simulink model "My_gfm_battery_sil_1_PPC2"  (R2018b)
settings: Solver=ode45  StartTime=0.0  StopTime=30  MaxStep=1e-4  RelTol=1e-3
PreLoadFcn:
  | modelDir = fileparts(get_param(bdroot,'FileName'));
  | 
  | load_system(fullfile(modelDir,'controls_element_lib.slx'));
  | load_system(fullfile(modelDir,'test_sequence_lib.slx'));
InitFcn:
  | close all;
  | clear all;
  | clc;
  | 
  | % frequency nominals
  | F_NOM = 60;
  | W_NOM = 2 * pi * F_NOM;
  | 
  | % base values relative to inverter
  | % --------------------------------
  | VLL_INV_NOM = 480;
  | P_INV_NOM = 1e6;
  | Q_INV_NOM = 0.5e6;
  | S_INV_NOM = sqrt(P_INV_NOM^2 + Q_INV_NOM^2);
  | 
  | I_INV_BASE = S_INV_NOM/(sqrt(3)*VLL_INV_NOM);
  | Z_INV_BASE = VLL_INV_NOM^2/S_INV_NOM;
  | L_INV_BASE = Z_INV_BASE / W_NOM;
  | C_INV_BASE = 1 / (Z_INV_BASE * W_NOM);
  | 
  | % nominal ratings for power system model
  | % --------------------------------------
  | INVERTER_COUNT = 100;
  | 
  | VLV_NOM = VLL_INV_NOM;
  | VMV_NOM = 35e3;
  | VHV_NOM = 230e3;
  | S_PLANT = INVERTER_COUNT * S_INV_NOM;
  | 
  | N_GSU = VHV_NOM/VMV_NOM;
  | N_MVT = VMV_NOM/VLV_NOM;
  | 
  | I_LV_BASE = S_PLANT/(sqrt(3)*VLV_NOM);
  | I_MV_BASE = S_PLANT/(sqrt(3)*VMV_NOM);
  | I_HV_BASE = S_PLANT/(sqrt(3)*VHV_NOM);
  | 
  | Z_LV_BASE = VLV_NOM^2/S_PLANT;
  | Z_MV_BASE = VMV_NOM^2/S_PLANT;
  | Z_HV_BASE = VHV_NOM^2/S_PLANT;
  | 
  | L_LV_BASE = Z_LV_BASE / W_NOM;
  | L_MV_BASE = Z_MV_BASE / W_NOM;
  | L_HV_BASE = Z_HV_BASE / W_NOM;
  | C_LV_BASE = 1 / (Z_LV_BASE * W_NOM);
  | C_MV_BASE = 1 / (Z_MV_BASE * W_NOM);
  | C_HV_BASE = 1 / (Z_HV_BASE * W_NOM);
undefined symbols (not defined in the file): dQmax, dQmin, dVmax, dVmin, j, vmax, vmin
libraries: simulink x54, test_sequence_lib x22, controls_element_lib x9
(part 1 of 7)
settings Model: SimulationMode=accelerator  Creator=HussamAlatrash  LastModifiedBy=ahhei
settings SolverCC: ZeroCrossAlgorithm=Adaptive
settings DataIOCC: ReturnWorkspaceOutputs=on
settings OptimizationCC: EfficientMapNaN2IntZero=off
settings DebuggingCC: IgnoredZcDiagnostic=none  UnconnectedInputMsg=none  UnconnectedOutputMsg=none  UnconnectedLineMsg=none
settings HardwareCC: TargetBitPerPointer=64  TargetBitPerSizeT=64  TargetBitPerPtrDiffT=64  TargetLongLongMode=on  TargetIntDivRoundTo=Zero  TargetEndianess=LittleEndian  TargetWordSize=64  TargetHWDeviceType=MATLAB Host  ProdEqTarget=off
settings ModelReferenceCC: EnableRefExpFcnMdlSchedulingChecks=off
settings CodeAppCC: MaxIdLength=128
settings GRTTargetCC: TargetLangStandard=C89/C90 (ANSI)  CombineOutputUpdateFcns=off  GRTInterface=on

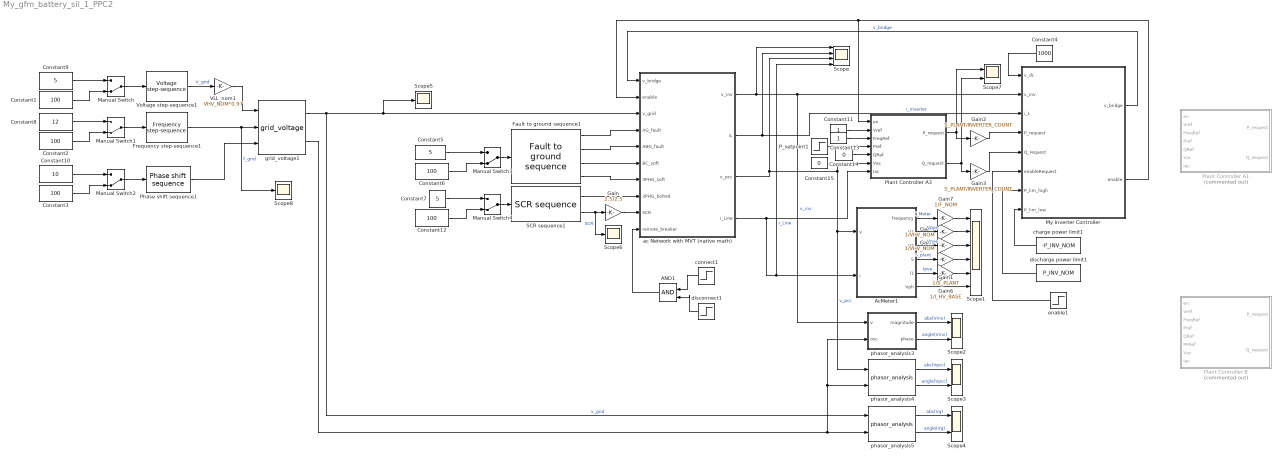
== system My_gfm_battery_sil_1_PPC2 ==
  AND1 : Logic  IconShape=distinctive  AllPortsSameDT=off  OutDataTypeStr=boolean
  AcMeter1 : Subsystem  AncestorBlock=test_sequence_lib/AcMeter  mask{VllRated=VHV_NOM}
      mask prompts: VllRated "Rated line voltage"
  Constant{1..3,6,12} (5 alike) : Constant  Value=100
  Constant10 : Constant  Value=10
  Constant11 : Constant
  Constant13 : Constant
  Constant14 : Constant  Value=0
  Constant15 : Constant  Value=0
  Constant4 : Constant  Value=1000
  Constant5 : Constant  Value=5
  Constant7 : Constant  Value=5
  Constant8 : Constant  Value=12
  Constant9 : Constant  Value=5
  Fault to ground sequence1 : test_sequence_lib/Fault to ground sequence  SystemSampleTime=-1
  Frequency step-sequence1 : test_sequence_lib/Frequency step-sequence  SystemSampleTime=-1
  Gain : Gain  Gain=2.5/2.5
  Gain1 : Gain  Gain=1/S_PLANT
  Gain2 : Gain  Gain=S_PLANT/INVERTER_COUNT
  Gain3 : Gain  Gain=S_PLANT/INVERTER_COUNT
  Gain4 : Gain  Gain=1/VHV_NOM
  Gain5 : Gain  Gain=1/VHV_NOM
  Gain6 : Gain  Gain=1/I_HV_BASE
  Gain7 : Gain  Gain=1/F_NOM
  Manual Switch{,1..4} (5 alike) : ManualSwitch  CurrentSetting=0
  "My Inverter Controller " : Subsystem
  P_setpoint1 : Step  Time=4  After=0.5  SampleTime=0
  Phase shift sequence1 : test_sequence_lib/Phase shift sequence  SystemSampleTime=-1
  Plant Controller A1 : Subsystem  Commented=on  mask(Renewable Energy Plant Controller (REPC_A)){Tfltr=0.02, Xc=0, Rc=0, Kc=0.04, db1=0, emax=0.2, emin=-0.2, Kp=1, Ki=5, Qmax=0.5, Qmin=-0.5, QRefmax=0.5, QRefmin=-0.5, Vfrz=0.8, Tft=0, Tfv=0.1, Vmax=1.05, Vmin=0.95, VcompMode=0, RPCMode=1, fdbd1=0.01*0, fdbd2=-0.01*0, Ddn=20, Dup=20, Tp=0.25, femax=1, femin=-1, Kpg=1, Kig=2, Tlag=0.2, Pmax=1.1, Pmin=-1.1, PRefmax=1, PRefmin=-1, Fmax=1.02, Fmin=-1.02, APCMode=1}
      mask prompts: Tfltr "Voltage/Reactive Power Time Constants [s]"; Xc "Line drop compensation reactance [pu]"; Rc "Line drop compensation resistance [pu]"; Kc "Reactive droop [pu]"; db1 "Reactive power deadline [pu]"; emax "Maximum Volt/VAR error [pu]"; emin "Minimum Volt/VAR error [pu]"; Kp "Volt/VAR Propotional Gain [pu/pu]"; Ki "Volt/VAR Integral Gain [pu/pu-s]"; Qmax "Max Cmd Reactive Power [pu]"; Qmin "Min Cmd Reactive Power [pu]"; QRefmax "Max Ref Reactive Power [pu]"; QRefmin "Min Ref Reactive Power [pu]"; Vfrz "Voltage for Freezing Volt/VAR Integrator [pu]"; Tft "Q Lead Time Constant [s]"; Tfv "Q Lag Time Constant [s]"; Vmax "Maximun Voltage Reference [pu]"; Vmin "Minimum Voltage Reference [pu]"; VcompMode "Voltage Compensation Mode"; RPCMode "Reactive Power Control Mode"; fdbd1 "Overfrequency deadband for govenor [pu]"; fdbd2 "Underfrequency deadband for govenor [pu]"; Ddn "Down regulation droop [pu]"; Dup "Up regulation droop [pu]"; Tp "Active Power Filter Time Constant [s]"; femax "Maximum Power Error [pu]"; femin "Minimum Power Error [pu]"; Kpg "Active Power regulator gain [pu]"; Kig "Active Power integral gain [pu]"; Tlag "Plant Controller P output Lag [s]"; Pmax "Maximum Cmd Active Power [pu]"; Pmin "Minimum Cmd Active Power [pu]"; PRefmax "Maximum Ref Active Power [pu]"; PRefmin "Minimum Ref Active Power [pu]"; Fmax "Maximum Frequency Reference [pu]"; Fmin "Minimum Frequency Reference [pu]"; APCMode "Active Power Control Mode"
      mask DialogControl Container3 Prompt: Reactive Power Control
      mask DialogControl Container4 Prompt: Active Power Control
  Plant Controller A3 : Subsystem  mask(Renewable Energy Plant Controller (REPC_A)){Tfltr=0.02, Xc=0, Rc=0, Kc=0.04, db1=0, emax=0.2, emin=-0.2, Kp=1, Ki=5, Qmax=0.5, Qmin=-0.5, QRefmax=0.5, QRefmin=-0.5, Vfrz=0.8, Tft=0, Tfv=0.1, Vmax=1.05, Vmin=0.95, VcompMode=0, RPCMode=1, fdbd1=0.01*0, fdbd2=-0.01*0, Ddn=20, Dup=20, Tp=0.25, femax=1, femin=-1, Kpg=1, Kig=2, Tlag=0.2, Pmax=1.1, Pmin=-1.1, PRefmax=1, PRefmin=-1, Fmax=1.02, Fmin=-1.02, APCMode=1}
      mask prompts: Tfltr "Voltage/Reactive Power Time Constants [s]"; Xc "Line drop compensation reactance [pu]"; Rc "Line drop compensation resistance [pu]"; Kc "Reactive droop [pu]"; db1 "Reactive power deadline [pu]"; emax "Maximum Volt/VAR error [pu]"; emin "Minimum Volt/VAR error [pu]"; Kp "Volt/VAR Propotional Gain [pu/pu]"; Ki "Volt/VAR Integral Gain [pu/pu-s]"; Qmax "Max Cmd Reactive Power [pu]"; Qmin "Min Cmd Reactive Power [pu]"; QRefmax "Max Ref Reactive Power [pu]"; QRefmin "Min Ref Reactive Power [pu]"; Vfrz "Voltage for Freezing Volt/VAR Integrator [pu]"; Tft "Q Lead Time Constant [s]"; Tfv "Q Lag Time Constant [s]"; Vmax "Maximun Voltage Reference [pu]"; Vmin "Minimum Voltage Reference [pu]"; VcompMode "Voltage Compensation Mode"; RPCMode "Reactive Power Control Mode"; fdbd1 "Overfrequency deadband for govenor [pu]"; fdbd2 "Underfrequency deadband for govenor [pu]"; Ddn "Down regulation droop [pu]"; Dup "Up regulation droop [pu]"; Tp "Active Power Filter Time Constant [s]"; femax "Maximum Power Error [pu]"; femin "Minimum Power Error [pu]"; Kpg "Active Power regulator gain [pu]"; Kig "Active Power integral gain [pu]"; Tlag "Plant Controller P output Lag [s]"; Pmax "Maximum Cmd Active Power [pu]"; Pmin "Minimum Cmd Active Power [pu]"; PRefmax "Maximum Ref Active Power [pu]"; PRefmin "Minimum Ref Active Power [pu]"; Fmax "Maximum Frequency Reference [pu]"; Fmin "Minimum Frequency Reference [pu]"; APCMode "Active Power Control Mode"
      mask DialogControl Container3 Prompt: Reactive Power Control
      mask DialogControl Container4 Prompt: Active Power Control
  Plant Controller B : Subsystem  Commented=on  mask(Renewable Energy Plant Controller (REPC_A)){Tfltr=0.02, Ts=1e-3, Vfrz=0.8, VcompMode=0, Kc=0.04, Vmax=1.05, Vmin=0.95, Verrmax=0.2, Verrmin=-0.2, vdbd1=0, vdbd2=0, Kpvdn=1, Kpvup=1, Tpv=0.1, Kiv=0, Vleak=10e-3, Vintmax=0.3, Vintmin=-0.3, RPCMode=1, Tpf=0, QRiseRate=1, QFallRate=-1, QRefmax=0.5, QRefmin=-0.5, Kpq=1, Kiq=2, Qleak=10e-3, Qerrmax=0.2, Qerrmin=-0.2, Qintmax=0.3, Qintmin=-0.3, Xc=0, Qmax=0.5, Qmin=-0.5, Tleadq=0, Tlagq=0.1, PRiseRate=1, PFallRate=-1, Fmax=1.05, Fmin=0.95, fdbd1=0.01*0, fdbd2=-0.01*0, Kpfdn=20, Kpfup=20, Pfreqmax=0.5, Pfreqmin=-0.5, Tfp=0.1, FFRLo_en=0, FFRThresLo=58.5/60, FFRTrigLoTime=0.2, FFRRestLo_en=0, FFRRestThresLo=59.5/60, FFRRestLoTime=0.2, FFRHoldLoTime=5, FFRPowerLo=0.5, FFRLoRiseRate=1, FFRLoFallRate=-1, Time1=0, FFRHi_en=0, FFRThresHi=61.5/60, FFRTrigHiTime=0.2, FFRRestHi_en=0, FFRRestThresHi=60.5/60, FFRRestHiTime=0.2, FFRHoldHiTime=5, FFRPowerHi=-0.5, FFRHiRiseRate=1, FFRHiFallRate=-1, Time2=0, PRefmax=1, PRefmin=-1, Tp=0.02, Kpp=1, Kip=2, Pleak=10e-3, Perrmax=0.2, Perrmin=-0.2, Pintmax=0.3, Pintmin=-0.3, APCMode=1, Rc=0, Pmax=1.1, Pmin=-1.1, Tlagp=0.2}
      mask prompts: Tfltr "Voltage/Reactive Power Time Constants [s]"; Ts "Time Step"; Vfrz "LVRT Threshold Voltage [pu]"; VcompMode "Voltage Compensation Mode"; Kc "Reactive droop [pu]"; Vmax "Maximum Voltage Reference [pu]"; Vmin "Minimum Voltage Reference [pu]"; Verrmax "Maximum Voltage Error  [pu]"; Verrmin "Minimum Voltage Error  [pu]"; vdbd1 "Voltage HiDeadband [pu]"; vdbd2 "Voltage LoDeadband [pu]"; Kpvdn "Voltage Down Proportional Gain [pu]"; Kpvup "Voltage Up Proportional Gain [pu]"; Tpv "Voltage Proportinal LPF Time Constants [s]"; Kiv "Voltage Integral Gain [pu]"; Vleak "Voltage Integral Leak Gain [pu]"; Vintmax "Maximum Voltage Integrator error [pu]"; Vintmin "Minimum Voltage Integrator error [pu]"; RPCMode "Reactive Power Control Mode"; Tpf "Power Factor LPF Time Constants [s]"; QRiseRate "Reactive Power Reference Rise Ramp Rate [pu/s]"; QFallRate "Reactive Power Reference Fall Ramp Rate [pu/s]"; QRefmax "Max Ref Reactive Power [pu]"; QRefmin "Min Ref Reactive Power [pu]"; Kpq "Reactive Power Propotional Gain [pu]"; Kiq "Reactive Power Integral Gain [pu]"; Qleak "Reactive Power Integral Leak Gain [pu]"; Qerrmax "Maximum Reactive Power error [pu]"; Qerrmin "Minimum Reactive Power error [pu]"; Qintmax "Maximum Reactive Power Integrator error [pu]"; Qintmin "Minimum Reactive Power Integrator error [pu]"; Xc "Loss compensation reactance [pu]"; Qmax "Max Cmd Reactive Power [pu]"; Qmin "Min Cmd Reactive Power [pu]"; Tleadq "Reactive Power Output Lead Time Constant [s]"; Tlagq "Reactive Power Output Lag Time Constant [s]"; PRiseRate "Active Power Reference Rise Ramp Rate [pu/s]"; PFallRate "Active Power Reference Fall Ramp Rate [pu/s]"; Fmax "Maximum Frequency Reference [pu]"; Fmin "Minimum Frequency Reference [pu]"; fdbd1 "Frequency HiDeadband [pu]"; fdbd2 "Frequency Lodeadband [pu]"; Kpfdn "Frequency Down Proportional Gain [pu]"; Kpfup "Frequency Up Proportional Gain [pu]"; Pfreqmax "Maximum Frequency Power [pu]"; Pfreqmin "Minimum Frequency Power [pu]"; Tfp "Frequency Power Proportinal LPF Time Constants [s]"; FFRLo_en "Enable Under Frequency FFR"; FFRThresLo "Trigger Threshold [pu]"; FFRTrigLoTime "Trigger Qualification Time [sec]"; FFRRestLo_en "Enable Restore Threshold"; FFRRestThresLo "Restore Threshold [pu]"; FFRRestLoTime "Restore Qualification Time [sec]"; FFRHoldLoTime "Hold Time [sec]"; FFRPowerLo "Power Response [pu]"; FFRLoRiseRate "Power Response Rise Rate [pu/s]"; FFRLoFallRate "Power Response Fall Rate [pu/s]"; Time1 "Condition Clear Time [sec]"; FFRHi_en "Enable Under Frequency FFR"; FFRThresHi "Trigger Threshold [pu]"; FFRTrigHiTime "Trigger Qualification Time [sec]"; FFRRestHi_en "Enable RestoreThreshold"; FFRRestThresHi "Restore Threshold [pu]"; FFRRestHiTime "Restore Qualification Time [sec]"; FFRHoldHiTime "Hold Time [sec]"; FFRPowerHi "Power Response [pu]"; FFRHiRiseRate "Power Response Rise Rate [pu/s]"; FFRHiFallRate "Power Response Fall Rate [pu/s]"; Time2 "Condition Clear Time [sec]"; PRefmax "Maximum Ref Active Power [pu]"; PRefmin "Minimum Ref Active Power [pu]"; Tp "Active Power Filter Time Constant [s]"; Kpp "Active Power Propotional Gain [pu]"; Kip "Active Power Integral Gain [pu]"; Pleak "Active Power Integral Leak Gain [pu]"; Perrmax "Maximum Active Power error [pu]"; Perrmin "Minimum Active Power error [pu]"; Pintmax "Maximum Active Power Integrator error [pu]"; Pintmin "Minimum Active Power Integrator error [pu]"; APCMode "Active Power Control Mode"; Rc "Loss compensation resistance [pu]"; Pmax "Maximum Cmd Active Power [pu]"; Pmin "Minimum Cmd Active Power [pu]"; Tlagp "Active Power Output Lag Time Constant [s]"
      mask DialogControl Container15 Prompt: Reactive Power Path
      mask DialogControl Container3 Prompt: Voltage/Reactive Power Control
      mask DialogControl Container5 Prompt: Voltage Control
      mask DialogControl Container6 Prompt: Reactive Power Control
      mask DialogControl Container20 Prompt: Active Power Path
      mask DialogControl Container4 Prompt: Reference and Control
      mask DialogControl Container9 Prompt: Active Power Reference
      mask DialogControl Container10 Prompt: Frequency Control
      mask DialogControl Container11 Prompt: Primary Frequency Response
      mask DialogControl Container13 Prompt: Fast Frequency Response
      mask DialogControl Container16 Prompt: Under Frequency FFR
      mask DialogControl Container16_copy Prompt: Over Frequency FFR
      mask DialogControl Container8 Prompt: Active Power Control
  SCR sequence1 : test_sequence_lib/SCR sequence  SystemSampleTime=-1
  Scope : Scope  NumInputPorts=4
  Scope1 : Scope  NumInputPorts=6
  Scope{2..4,7} (4 alike) : Scope  NumInputPorts=2
  Scope5 : Scope
  Scope6 : Scope
  Scope8 : Scope
  VLL_nom1 : Gain  Gain=VHV_NOM*0.97
  Voltage step-sequence1 : test_sequence_lib/Voltage step-sequence  SystemSampleTime=-1
  ac Network with MVT (native math) : Subsystem  AncestorBlock=test_sequence_lib/ac Network with MVT (native math)
  charge power limit1 : Constant  Value=-P_INV_NOM
  connect1 : Step  Time=0  SampleTime=0
  discharge power limit1 : Constant  Value=P_INV_NOM
  disconnect1 : Step  Time=100  Before=1  After=0  SampleTime=0
  enable1 : Step  Time=0.5  SampleTime=0
  grid_voltage1 : test_sequence_lib/grid_voltage  SystemSampleTime=-1
  phasor_analysis3 : Subsystem  AncestorBlock=test_sequence_lib/phasor_analysis
  phasor_analysis4 : test_sequence_lib/phasor_analysis  SystemSampleTime=-1
  phasor_analysis5 : test_sequence_lib/phasor_analysis  SystemSampleTime=-1
  wires:
  Voltage step-sequence1/1 -> VLL_nom1/1  "V_grid"
  Manual Switch/1 -> Voltage step-sequence1/1
  Fault to ground sequence1/2 -> ac Network with MVT (native math)/5(ABG_fault)
  AND1/1 -> ac Network with MVT (native math)/10(remote_breaker)
  Constant4/1 -> "My Inverter Controller "/1(v_dc)
  AcMeter1/3(V2) -> Gain5/1  "Vnve"
  discharge power limit1/1 -> "My Inverter Controller "/7(P_lim_high)
  Fault to ground sequence1/3 -> ac Network with MVT (native math)/6(BC_soft)
  AcMeter1/6(Vph) -> Scope1/6
  "My Inverter Controller "/1(v_bridge) -> ac Network with MVT (native math)/1(v_bridge)  "v_bridge"
  AcMeter1/2(V1) -> Gain4/1  "Vpve"
  Plant Controller A3/1(P_request) -> Gain2/1, Scope7/1
  ac Network with MVT (native math)/1(v_inv) -> phasor_analysis3/1(v), "My Inverter Controller "/2(v_inv), Scope/1  "v_inv"
  phasor_analysis5/1 -> Scope4/1  "abs(Vg)"
  AcMeter1/5(I1) -> Gain6/1  "Ipve"
  Plant Controller A3/2(Q_request) -> Gain3/1, Scope7/2
  grid_voltage1/1 -> phasor_analysis5/1, Scope5/1, ac Network with MVT (native math)/3(v_grid)  "v_grid"
  SCR sequence1/1 -> ac Network with MVT (native math)/8(3PHG_bolted)
  phasor_analysis3/1(magnitude) -> Scope2/1  "abs(Vinv)"
  AcMeter1/4(S) -> Gain1/1  "S_plant"
  ac Network with MVT (native math)/4(i_Line) -> Plant Controller A3/7(Iac), Scope/4, AcMeter1/2(i)  "i_Line"
  AcMeter1/1(frequency) -> Gain7/1  "f_Meter"
  VLL_nom1/1 -> grid_voltage1/1
  phasor_analysis3/2(phase) -> Scope2/2  "angle(Vinv)"
  SCR sequence1/2 -> Scope6/1, Gain/1  "SCR"
  ac Network with MVT (native math)/2(iL) -> "My Inverter Controller "/3(i_L), Scope/2  "i_inverter"
  disconnect1/1 -> AND1/2
  Fault to ground sequence1/4 -> ac Network with MVT (native math)/7(3PHG_soft)
  ac Network with MVT (native math)/3(v_pcc) -> Plant Controller A3/6(Vac), phasor_analysis4/1, AcMeter1/1(v), Scope/3  "v_pcc"
  charge power limit1/1 -> "My Inverter Controller "/8(P_lim_low)
  "My Inverter Controller "/2(enable) -> Plant Controller A3/1(en), ac Network with MVT (native math)/2(enable)
  Frequency step-sequence1/1 -> Scope8/1, grid_voltage1/2  "f_grid"
  Fault to ground sequence1/1 -> ac Network with MVT (native math)/4(AG_fault)
  grid_voltage1/2 -> phasor_analysis4/2, phasor_analysis3/2(osc), phasor_analysis5/2
  phasor_analysis5/2 -> Scope4/2  "angle(Vg)"
  enable1/1 -> "My Inverter Controller "/6(enableRequest)
  connect1/1 -> AND1/1
  Constant9/1 -> Manual Switch/1
  Constant1/1 -> Manual Switch/2
  Constant2/1 -> Manual Switch1/2
  Manual Switch1/1 -> Frequency step-sequence1/1
  Constant8/1 -> Manual Switch1/1
  Manual Switch2/1 -> Phase shift sequence1/1
  Constant3/1 -> Manual Switch2/2
  Constant10/1 -> Manual Switch2/1
  Constant6/1 -> Manual Switch3/2
  Constant5/1 -> Manual Switch3/1
  Manual Switch3/1 -> Fault to ground sequence1/1
  Constant7/1 -> Manual Switch4/1
  Constant12/1 -> Manual Switch4/2
  Manual Switch4/1 -> SCR sequence1/1
  phasor_analysis4/1 -> Scope3/1  "abs(Vpcc)"
  phasor_analysis4/2 -> Scope3/2  "angle(Vpcc)"
  Phase shift sequence1/1 -> grid_voltage1/3
  Gain2/1 -> "My Inverter Controller "/4(P_request)
  Gain3/1 -> "My Inverter Controller "/5(Q_request)
  Gain/1 -> ac Network with MVT (native math)/9(SCR)
  Gain1/1 -> Scope1/4
  Gain4/1 -> Scope1/2
  Gain5/1 -> Scope1/3
  Gain6/1 -> Scope1/5
  Gain7/1 -> Scope1/1
  Constant11/1 -> Plant Controller A3/2(Vref)
  Constant13/1 -> Plant Controller A3/3(FreqRef)
  P_setpoint1/1 -> Plant Controller A3/4(Pref)
  Constant14/1 -> Plant Controller A3/5(QRef)

== system My_gfm_battery_sil_1_PPC2/AcMeter1 ==
  note: in pu:
      | S = sqrt(3) * VLL * conj(I)
  v : Inport
  i : Inport  Port=2
  Complex to Magnitude : ComplexToMagnitudeAngle  Output=Magnitude
  Complex to Magnitude1 : ComplexToMagnitudeAngle  Output=Magnitude
  Complex to Magnitude2 : ComplexToMagnitudeAngle  Output=Magnitude
  Conj : Math  Operator=conj  SaturateOnIntegerOverflow=on
  PLL_3ph : Subsystem
  Product : Product
  RMS calculator : Subsystem
  Sum of Elements : Sum  Inputs=+
  Terminator : Terminator
  Terminator1 : Terminator
  Terminator2 : Terminator
  overVnom : Gain  Gain=1/VllRated
  phasor_analysis : Subsystem
  phasor_analysis1 : Subsystem  AncestorBlock=test_sequence_lib/AcMeter/phasor_analysis
  sqrt(3) : Gain  Gain=sqrt(3)
  sqrt(3)1 : Gain  Gain=sqrt(3)
  sqrt(3)2 : Gain  Gain=sqrt(3)
  frequency : Outport  VectorParamsAs1DForOutWhenUnconnected=on
  V1 : Outport  Port=2  VectorParamsAs1DForOutWhenUnconnected=on
  V2 : Outport  Port=3  VectorParamsAs1DForOutWhenUnconnected=on
  S : Outport  Port=4  VectorParamsAs1DForOutWhenUnconnected=on
  I1 : Outport  Port=5  VectorParamsAs1DForOutWhenUnconnected=on
  Vph : Outport  Port=6  VectorParamsAs1DForOutWhenUnconnected=on
  wires:
  RMS calculator/1(out[3]) -> Vph/1
  PLL_3ph/2(osc[3]) -> phasor_analysis/2(osc), phasor_analysis1/2(osc)
  Sum of Elements/1 -> S/1  "S"
  v/1 -> RMS calculator/1(in[3]), phasor_analysis/1(in), overVnom/1
  PLL_3ph/1(freq) -> frequency/1
  overVnom/1 -> PLL_3ph/1(ref)
  Conj/1 -> Product/2
  Product/1 -> Sum of Elements/1
  phasor_analysis/2(pve) -> sqrt(3)/1  "Vpve_LN"
  phasor_analysis/3(nve) -> sqrt(3)1/1
  phasor_analysis1/2(pve) -> Complex to Magnitude2/1, Conj/1  "Ipve"
  sqrt(3)1/1 -> Complex to Magnitude1/1  "Vnve_LL"
  i/1 -> phasor_analysis1/1(in)
  sqrt(3)/1 -> Complex to Magnitude/1, sqrt(3)2/1  "Vpve_LL"
  sqrt(3)2/1 -> Product/1
  phasor_analysis/1(perPh) -> Terminator/1
  phasor_analysis1/1(perPh) -> Terminator1/1
  phasor_analysis1/3(nve) -> Terminator2/1
  Complex to Magnitude/1 -> V1/1  "Ve"
  Complex to Magnitude1/1 -> V2/1  "Ve"
  Complex to Magnitude2/1 -> I1/1  "Ve"

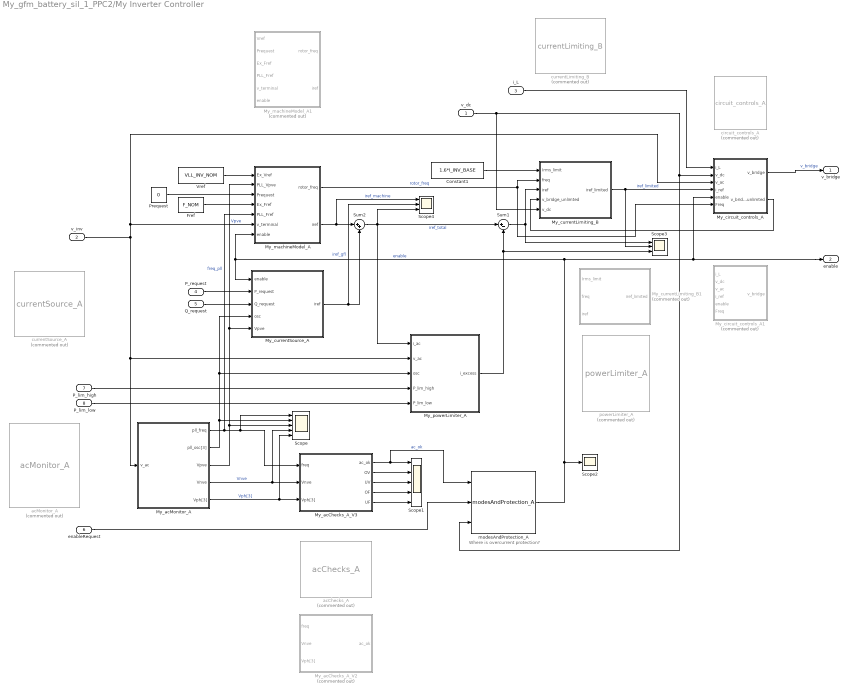
== system My_gfm_battery_sil_1_PPC2/My Inverter Controller  ==
  note: Where is overcurrent protection?
  v_dc : Inport
  v_inv : Inport  Port=2
  i_L : Inport  Port=3
  P_request : Inport  Port=4
  Q_request : Inport  Port=5
  enableRequest : Inport  Port=6
  P_lim_high : Inport  Port=7
  P_lim_low : Inport  Port=8
  Constant1 : Constant  Value=1.6*I_INV_BASE
  Fref : Constant  Value=F_NOM
  My_acChecks_A_V2 : Subsystem  Commented=on  AncestorBlock=controls_element_lib/acChecks_A  mask{VllRated=VLL_INV_NOM, NominalFrequency=F_NOM, Ts=1e-3, Time1=2, Time2=0, VHi=1.15, VLo=0.85, FHi=62, FLo=58, VNeg=0.2, Time3=0, OV3=1.3, OV3_Time=0.02, OV3_en=1, OV2=1.25, OV2_Time=2, OV2_en=1, OV1=1.2, OV1_Time=20, OV1_en=1, UV1=0.81, UV1_Time=15, UV1_en=1, UV2=0.5, UV2_Time=5, UV2_en=1, UV3=0.2, UV3_Time=1, UV3_en=1, OF3=70, OF3_Time=0.2, OF3_en=1, OF2=65, OF2_Time=10, OF2_en=1, OF1=63, OF1_Time=30, OF1_en=1, UF1=56, UF1_Time=30, UF1_en=1, UF2=55, UF2_Time=10, UF2_en=1, UF3=50, UF3_Time=0.2, UF3_en=1}
      mask prompts: VllRated "Rated Line-to-Line Voltage (V)"; NominalFrequency "Nominal Line Frequency (Hz)"; Ts "Operating Sample Time (sec)"; Time1 "Connection Time (sec)"; Time2 "Connection Out-of-Condition Delay (sec)"; VHi "High Voltage Threshold (pu)"; VLo "Low Voltage Threshold (pu)"; FHi "High Frequency Threshold (Hz)"; FLo "Low Frequency Threshold (Hz)"; VNeg "Negative Sequence Voltage Threshold (pu)"; Time3 "Trip Out-of-Condition Delay (sec)"; OV3 "OV PickUp 3 (pu)"; OV3_Time "OV Time 3 (sec)"; OV3_en "OV Enable 3"; OV2 "OV PickUp 2 (pu)"; OV2_Time "OV Time 2 (sec)"; OV2_en "OV Enable 2"; OV1 "OV PickUp 1 (pu)"; OV1_Time "OV Time 1 (sec)"; OV1_en "OV Enable 1"; UV1 "UV PickUp 1 (pu)"; UV1_Time "UV Time 1 (sec)"; UV1_en "UV Enable 1"; UV2 "UV PickUp 2 (pu)"; UV2_Time "UV Time 2 (sec)"; UV2_en "UV Enable 2"; UV3 "UV PickUp 3 (pu)"; UV3_Time "UV Time 3 (sec)"; UV3_en "UV Enable 3"; OF3 "OF PickUp 3 (Hz)"; OF3_Time "OF Time 3 (pu)"; OF3_en "OF Enable 3"; OF2 "OF PickUp 2 (Hz)"; OF2_Time "OF Time 2 (pu)"; OF2_en "OF Enable 2"; OF1 "OF PickUp 1 (Hz)"; OF1_Time "OF Time 1 (pu)"; OF1_en "OF Enable 1"; UF1 "UF PickUp 1 (Hz)"; UF1_Time "UF Time 1 (sec)"; UF1_en "UF Enable 1"; UF2 "UF PickUp 2 (Hz)"; UF2_Time "UF Time 2 (sec)"; UF2_en "UF Enable 2"; UF3 "UF PickUp 3 (Hz)"; UF3_Time "UF Time 3 (sec)"; UF3_en "UF Enable 3"
      mask DialogControl DescGroupVar Prompt: ACChecks
      mask DialogControl DecsTextVar Prompt: Grid Checks for Connection and Tripping
      mask DialogControl ParameterGroupVar Prompt: General Parameters
      mask DialogControl Container11 Prompt: Connection Settings
      mask DialogControl Container20 Prompt: Thresholds
      mask DialogControl Container3 Prompt: Trip Settings
      mask DialogControl Container12 Prompt: General Parameters
      mask DialogControl Container15 Prompt: Over Voltage Settings
      mask DialogControl Container4 Prompt: Over Voltage
      mask DialogControl Container19 Prompt: Under Voltage Settings
      mask DialogControl Container7 Prompt: Under Voltage
      mask DialogControl Container17 Prompt: Over Frequency Settings
      mask DialogControl Container9 Prompt: Over Frequency
      mask DialogControl Container16 Prompt: Under Frequency Settings
      mask DialogControl Container10 Prompt: Under Frequency
  My_acChecks_A_V3 : Subsystem  AncestorBlock=controls_element_lib/acChecks_A  mask{VllRated=VLL_INV_NOM, NominalFrequency=F_NOM, Ts=1e-3, Time1=2, Time2=0, VHi=1.15, VLo=0.85, FHi=62, FLo=58, VNeg=0.2, Time3=0, OV3=1.3, OV3_Time=0.02, OV3_en=1, OV2=1.25, OV2_Time=2, OV2_en=1, OV1=1.2, OV1_Time=20, OV1_en=1, UV1=0.81, UV1_Time=15, UV1_en=1, UV2=0.5, UV2_Time=5, UV2_en=1, UV3=0.2, UV3_Time=1, UV3_en=1, OF3=70, OF3_Time=0.2, OF3_en=1, OF2=65, OF2_Time=10, OF2_en=1, OF1=63, OF1_Time=30, OF1_en=1, UF1=56, UF1_Time=30, UF1_en=1, UF2=55, UF2_Time=10, UF2_en=1, UF3=50, UF3_Time=0.2, UF3_en=1}
      mask prompts: VllRated "Rated Line-to-Line Voltage (V)"; NominalFrequency "Nominal Line Frequency (Hz)"; Ts "Operating Sample Time (sec)"; Time1 "Connection Time (sec)"; Time2 "Connection Out-of-Condition Delay (sec)"; VHi "High Voltage Threshold (pu)"; VLo "Low Voltage Threshold (pu)"; FHi "High Frequency Threshold (Hz)"; FLo "Low Frequency Threshold (Hz)"; VNeg "Negative Sequence Voltage Threshold (pu)"; Time3 "Trip Out-of-Condition Delay (sec)"; OV3 "OV PickUp 3 (pu)"; OV3_Time "OV Time 3 (sec)"; OV3_en "OV Enable 3"; OV2 "OV PickUp 2 (pu)"; OV2_Time "OV Time 2 (sec)"; OV2_en "OV Enable 2"; OV1 "OV PickUp 1 (pu)"; OV1_Time "OV Time 1 (sec)"; OV1_en "OV Enable 1"; UV1 "UV PickUp 1 (pu)"; UV1_Time "UV Time 1 (sec)"; UV1_en "UV Enable 1"; UV2 "UV PickUp 2 (pu)"; UV2_Time "UV Time 2 (sec)"; UV2_en "UV Enable 2"; UV3 "UV PickUp 3 (pu)"; UV3_Time "UV Time 3 (sec)"; UV3_en "UV Enable 3"; OF3 "OF PickUp 3 (Hz)"; OF3_Time "OF Time 3 (pu)"; OF3_en "OF Enable 3"; OF2 "OF PickUp 2 (Hz)"; OF2_Time "OF Time 2 (pu)"; OF2_en "OF Enable 2"; OF1 "OF PickUp 1 (Hz)"; OF1_Time "OF Time 1 (pu)"; OF1_en "OF Enable 1"; UF1 "UF PickUp 1 (Hz)"; UF1_Time "UF Time 1 (sec)"; UF1_en "UF Enable 1"; UF2 "UF PickUp 2 (Hz)"; UF2_Time "UF Time 2 (sec)"; UF2_en "UF Enable 2"; UF3 "UF PickUp 3 (Hz)"; UF3_Time "UF Time 3 (sec)"; UF3_en "UF Enable 3"
      mask DialogControl DescGroupVar Prompt: ACChecks
      mask DialogControl DecsTextVar Prompt: Grid Checks for Connection and Tripping
      mask DialogControl ParameterGroupVar Prompt: General Parameters
      mask DialogControl Container11 Prompt: Connection Settings
      mask DialogControl Container20 Prompt: Thresholds
      mask DialogControl Container3 Prompt: Trip Settings
      mask DialogControl Container12 Prompt: General Parameters
      mask DialogControl Container15 Prompt: Over Voltage Settings
      mask DialogControl Container4 Prompt: Over Voltage
      mask DialogControl Container19 Prompt: Under Voltage Settings
      mask DialogControl Container7 Prompt: Under Voltage
      mask DialogControl Container17 Prompt: Over Frequency Settings
      mask DialogControl Container9 Prompt: Over Frequency
      mask DialogControl Container16 Prompt: Under Frequency Settings
      mask DialogControl Container10 Prompt: Under Frequency
  My_acMonitor_A : Subsystem  AncestorBlock=controls_element_lib/acMonitor_A  mask{VllRated=VLL_INV_NOM, nominalFrequency=F_NOM}
      mask prompts: VllRated "Rated line-to-line voltage (V)"; nominalFrequency "Nominal line frequency (Hz)"
  My_circuit_controls_A : Subsystem  AncestorBlock=controls_element_lib/circuit_controls_A
  My_circuit_controls_A1 : Subsystem  Commented=on  AncestorBlock=controls_element_lib/circuit_controls_A
  My_currentLimiting_B : Subsystem  AncestorBlock=controls_element_lib/currentLimiting_B  mask{IRated=I_INV_BASE, peakSoftLimit=2.6, peakHardLimit=3.6}
      mask prompts: IRated "Rated current (A)"; peakSoftLimit "Soft peak limit (pu)"; peakHardLimit "Hard peak limit (pu)"
  My_currentLimiting_B1 : Subsystem  Commented=on  AncestorBlock=controls_element_lib/currentLimiting_B  mask{IRated=I_INV_BASE, peakSoftLimit=2.6, peakHardLimit=3.6}
      mask prompts: IRated "Rated current (A)"; peakSoftLimit "Soft peak limit (pu)"; peakHardLimit "Hard peak limit (pu)"
  My_currentSource_A : Subsystem  AncestorBlock=controls_element_lib/currentSource_A  mask{VllRated=VLL_INV_NOM, SRated=S_INV_NOM, nominalFrequency=F_NOM, Plimit=P_INV_NOM/S_INV_NOM, Qlimit=Q_INV_NOM/S_INV_NOM, CSOnline=1}
      mask prompts: VllRated "Rated line-to-line voltage (V)"; SRated "Rated power (VA)"; nominalFrequency "Nominal line frequency (Hz)"; Plimit "Real power request limit (pu)"; Qlimit "Reactive power request limit (pu)"; CSOnline "Current Source Online"
  My_machineModel_A : Subsystem  AncestorBlock=controls_element_lib/machineModel_A  mask{SRated=S_INV_NOM, VllRated=VLL_INV_NOM, nominalFrequency=F_NOM, MachOnline=0, inertialConstant=2.5, kDamper=2, tau_damp=0.3, Xs=0.3, rs=0.08, rn=0, wExciter=10, VoltRefSel=0, AVROnline=0, kqDroop=0, Xcomp=0, kp=5, ki=1, leak=10e-3, FreqRefSel=0, kDroop=1, wGoverner=1/0.3, kpSync=20, kpFastSync=1, wSync=2*pi*50, kpSyncFade=4, SyncFadeThres=0.2, tauMeas=0.02, tauBkSt=0.5}
      mask prompts: SRated "Rated power (VA)"; VllRated "Rated Voltage (Volts, line-to-line)"; nominalFrequency "Nominal frequency (Hz)"; MachOnline "Machine Online"; inertialConstant "Inertial constant (seconds)"; kDamper "Damper gain (pu/Hz)"; tau_damp "Damper time constant (sec)"; Xs "Stator reactance (pu)"; rs "Stator resistance (pu)"; rn "Neutral resistance (pu)"; wExciter "Exciter Bandwidth (rad)"; VoltRefSel "Voltage Reference Selector"; AVROnline "AVR Online"; kqDroop "QV Droop (pu v/ pu Q)"; Xcomp "Line drop compensation (pu)"; kp "Proportional gain"; ki "Integral gain"; leak "Leakage"; FreqRefSel "Frequency Reference Selector"; kDroop "Droop gain (pu/Hz)"; wGoverner "Governer Bandwidth (rad/s)"; kpSync "Synchronizer proportional gain (pu P / pu V)"; kpFastSync "Fast synchronizer gain (pu P / pu V)"; wSync "Synchronizer HPF Bandwidth(rad/s)"; kpSyncFade "Synchronizer fade gain (pu P/ puV)"; SyncFadeThres "Synchronizer fade threshold (pu)"; tauMeas "Measurements filters time constant (sec)"; tauBkSt "Black Start filter time constant (sec)"
      mask DialogControl DescGroupVar Prompt: Machine Model and Controls
      mask DialogControl ParameterGroupVar Prompt: Ratings
      mask DialogControl Container3 Prompt: Machine Parameters
      mask DialogControl Container4 Prompt: Mechanical Parameters
      mask DialogControl Container5 Prompt: Electrical Parameters
      mask DialogControl Container7 Prompt: AVR Parameters
      mask DialogControl Container6 Prompt: Governer Parameters
      mask DialogControl Container9 Prompt: Synchronizer Parameters
  My_machineModel_A1 : Subsystem  Commented=on  AncestorBlock=controls_element_lib/machineModel_A  mask{SRated=S_INV_NOM, VllRated=VLL_INV_NOM, nominalFrequency=F_NOM, inertialConstant=2.5, kDroop=1, kDamper=2, Xs=0.3, rs=0.08, Qlimit1=0.5, wExciter=10, FreqRefSel=1, MachOnline=0}
      mask prompts: SRated "Rated power (VA)"; VllRated "Rated Voltage (Volts, line-to-line)"; nominalFrequency "Nominal frequency (Hz)"; inertialConstant "Inertial constant (seconds)"; kDroop "Droop gain (pu/Hz)"; kDamper "Damper gain (pu/Hz)"; Xs "Stator reactance (pu)"; rs "Stator resistance (pu)"; Qlimit1 "Reactive power request limit (pu)"; wExciter "Exciter Bandwidth (rad)"; FreqRefSel "Frequency Reference Selector"; MachOnline "Machine Online"
      mask DialogControl DescGroupVar Prompt: Machine Model and Controls
  My_powerLimiter_A : Subsystem  AncestorBlock=controls_element_lib/powerLimiter_A  mask{VllRated=VLL_INV_NOM, nominalFrequency=F_NOM, wPowerLimiter=3}
      mask prompts: VllRated "Rated line-to-line voltage (V)"; nominalFrequency "Nominal line frequency (Hz)"; wPowerLimiter "Bandwidth (rad)"
  Prequest : Constant  Value=0
  Scope : Scope  NumInputPorts=5
  Scope1 : Scope  NumInputPorts=5
  Scope2 : Scope
  Scope3 : Scope  NumInputPorts=3
  Scope4 : Scope  NumInputPorts=3
  Sum1 : Sum  Inputs=|+-
  Sum2 : Sum  Inputs=|++
  Vref : Constant  Value=VLL_INV_NOM
  acChecks_A : controls_element_lib/acChecks_A  Commented=on  VllRated=VLL_INV_NOM  nominalFrequency=F_NOM  tRequalify=2  T_CNTL=1e-3
  acMonitor_A : controls_element_lib/acMonitor_A  Commented=on  VllRated=VLL_INV_NOM  nominalFrequency=F_NOM
  circuit_controls_A : controls_element_lib/circuit_controls_A  Commented=on  SystemSampleTime=-1
  currentLimiting_B : controls_element_lib/currentLimiting_B  Commented=on  IRated=I_INV_BASE  peakSoftLimit=2.6  peakHardLimit=3.6
  currentSource_A : controls_element_lib/currentSource_A  Commented=on  VllRated=VLL_INV_NOM  SRated=S_INV_NOM  nominalFrequency=F_NOM  Plimit=P_INV_NOM/S_INV_NOM  Qlimit=Q_INV_NOM/S_INV_NOM
  modesAndProtection_A : controls_element_lib/modesAndProtection_A  dcOvervotlageThreshold=1800  dcUndervotlageThreshold=700  dcTripClearTimeout=0.2
  powerLimiter_A : controls_element_lib/powerLimiter_A  Commented=on  VllRated=VLL_INV_NOM  nominalFrequency=F_NOM  wPowerLimiter=3
  v_bridge : Outport  VectorParamsAs1DForOutWhenUnconnected=on
  enable : Outport  Port=2  VectorParamsAs1DForOutWhenUnconnected=on
  wires:
  Vref/1 -> My_machineModel_A/1(Ex_Vref)
  Prequest/1 -> My_machineModel_A/3(Prequest)
  My_machineModel_A/2(iref) -> Scope4/1, Sum2/1  "iref_machine"
  My_acMonitor_A/2(pll_osc[3]) -> Scope/2, My_currentSource_A/4(osc), My_powerLimiter_A/3(osc)
  My_currentLimiting_B/1(iref_limited) -> My_circuit_controls_A/4(i_ref), Scope3/2  "iref_limited"
  My_currentSource_A/1(iref) -> Sum2/2, Scope4/2  "iref_gfl"
  Sum2/1 -> Sum1/1, Scope4/3, My_powerLimiter_A/1(i_ac)  "iref_total"
  My_acMonitor_A/3(Vpve) -> My_machineModel_A/2(PLL_Vpve), My_currentSource_A/5(Vpve), Scope/3  "Vpve"
  Q_request/1 -> My_currentSource_A/3(Q_request)
  P_request/1 -> My_currentSource_A/2(P_request)
  enableRequest/1 -> modesAndProtection_A/2
  modesAndProtection_A/1 -> Scope2/1, My_machineModel_A/7(enable), My_currentSource_A/1(enable), My_circuit_controls_A/5(enable), enable/1  "enable"
  My_acMonitor_A/5(Vph[3]) -> My_acChecks_A_V3/3(Vph[3]), Scope/5  "Vph[3]"
  My_acChecks_A_V3/1(ac_ok) -> Scope1/1, modesAndProtection_A/1  "ac_ok"
  Constant1/1 -> My_currentLimiting_B/1(Irms_limit)
  My_acMonitor_A/1(pll_freq) -> My_machineModel_A/5(PLL_Fref), My_acChecks_A_V3/1(freq), Scope/1  "freq_pll"
  My_acMonitor_A/4(Vnve) -> My_acChecks_A_V3/2(Vnve), Scope/4  "Vnve"
  P_lim_low/1 -> My_powerLimiter_A/5(P_lim_low)
  P_lim_high/1 -> My_powerLimiter_A/4(P_lim_high)
  My_powerLimiter_A/1(i_excess) -> Sum1/2, Scope3/3
  Sum1/1 -> My_currentLimiting_B/3(iref), Scope3/1
  v_dc/1 -> My_circuit_controls_A/2(v_dc), modesAndProtection_A/3, My_currentLimiting_B/5(v_dc)
  My_circuit_controls_A/1(v_bridge) -> v_bridge/1  "v_bridge"
  My_machineModel_A/1(rotor_freq) -> My_circuit_controls_A/6(Freq), My_currentLimiting_B/2(freq)  "rotor_freq"
  i_L/1 -> My_circuit_controls_A/1(i_L)
  v_inv/1 -> My_circuit_controls_A/3(v_ac), My_machineModel_A/6(v_terminal), My_acMonitor_A/1(v_ac), My_powerLimiter_A/2(v_ac)
  Fref/1 -> My_machineModel_A/4(Ex_Fref)
  My_acChecks_A_V3/2(OV) -> Scope1/2
  My_acChecks_A_V3/3(UV) -> Scope1/3
  My_acChecks_A_V3/4(OF) -> Scope1/4
  My_acChecks_A_V3/5(UF) -> Scope1/5
  My_circuit_controls_A/2(v_bridge_unlimted) -> My_currentLimiting_B/4(v_bridge_unlimted)

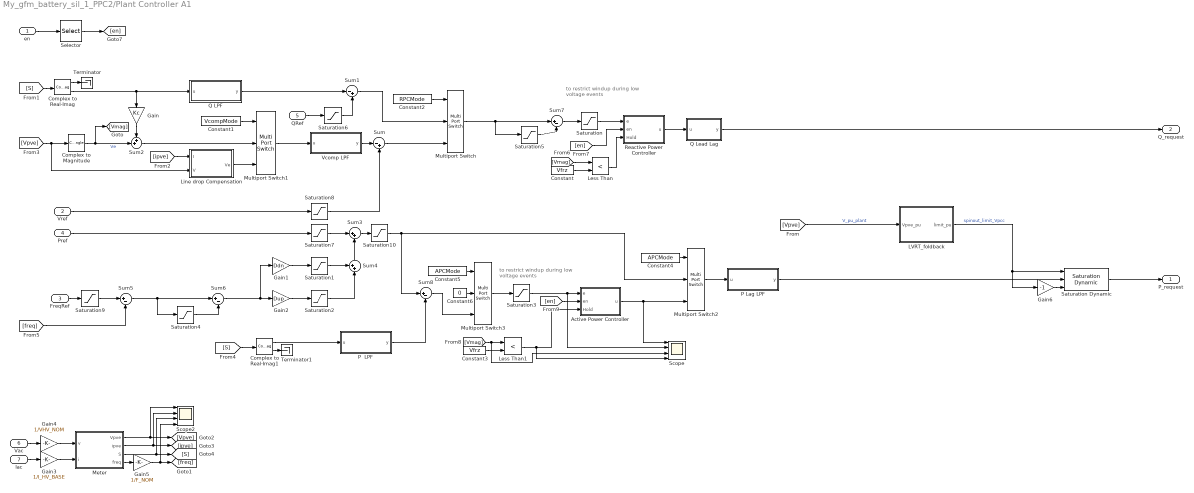
== system My_gfm_battery_sil_1_PPC2/Plant Controller A1 ==
  note: to restrict windup
      | during low voltage events
  note: to restrict windup
      | during low voltage events
  en : Inport
  Vref : Inport  Port=2
  FreqRef : Inport  Port=3
  Pref : Inport  Port=4
  QRef : Inport  Port=5
  Vac : Inport  Port=6
  Iac : Inport  Port=7
  Active Power Controller : Subsystem
  Complex to Real-Imag : ComplexToRealImag
  Complex to Real-Imag1 : ComplexToRealImag
  Complex to Magnitude : ComplexToMagnitudeAngle  Output=Magnitude
  Constant : Constant  Value=Vfrz
  Constant1 : Constant  Value=VcompMode
  Constant2 : Constant  Value=RPCMode
  Constant3 : Constant  Value=Vfrz
  Constant4 : Constant  Value=APCMode
  Constant5 : Constant  Value=APCMode
  Constant6 : Constant  Value=0
  Gain : Gain  Gain=Kc
  Gain1 : Gain  Gain=Ddn
  Gain2 : Gain  Gain=Dup
  Gain3 : Gain  Gain=1/I_HV_BASE
  Gain4 : Gain  Gain=1/VHV_NOM
  Gain5 : Gain  Gain=1/F_NOM
  Gain6 : Gain  Gain=-1
  LVRT_foldback : Subsystem
  Less Than : RelationalOperator  Operator=<  OutDataTypeStr=boolean  RndMeth=Simplest
  Less Than1 : RelationalOperator  Operator=<  OutDataTypeStr=boolean  RndMeth=Simplest
  Line drop Compensation : Subsystem
  Meter : Subsystem
  Multiport Switch{,1..3} (4 alike) : MultiPortSwitch  DataPortOrder=Zero-based contiguous  Inputs=2  zeroidx=on
  P  LPF : Subsystem
  P Lag LPF : Subsystem
  Q LPF : Subsystem
  Q Lead Lag : Subsystem
  Reactive Power Controller : Subsystem
  Saturation : Saturate  UpperLimit=emax  LowerLimit=emin
  Saturation Dynamic : simulink/Discontinuities/Saturation Dynamic  OutMin=[]  OutMax=[]  OutDataTypeStr=Inherit: Same as second input  OutDataType=fixdt(1, 16)  OutScaling=2^-10  DoSatur=off
  Saturation1 : Saturate  UpperLimit=0  LowerLimit=-inf
  Saturation10 : Saturate  UpperLimit=PRefmax  LowerLimit=PRefmin
  Saturation2 : Saturate  UpperLimit=inf  LowerLimit=0
  Saturation3 : Saturate  UpperLimit=femax  LowerLimit=femin
  Saturation4 : Saturate  UpperLimit=fdbd1  LowerLimit=fdbd2
  Saturation5 : Saturate  UpperLimit=db1  LowerLimit=-db1
  Saturation6 : Saturate  UpperLimit=QRefmax  LowerLimit=QRefmin
  Saturation7 : Saturate  UpperLimit=PRefmax  LowerLimit=PRefmin
  Saturation8 : Saturate  UpperLimit=Vmax  LowerLimit=Vmin
  Saturation9 : Saturate  UpperLimit=Fmax  LowerLimit=Fmin
  Scope : Scope  NumInputPorts=4
  Scope2 : Scope  NumInputPorts=4
  Selector : Selector  InputPortWidth=3  IndexOptions=Index vector (dialog)  Indices=[1]  OutputSizes=1
  Sum : Sum  Inputs=|-+
  Sum1 : Sum  Inputs=|-+
  Sum2 : Sum  Inputs=++|
  Sum3 : Sum  Inputs=|++
  Sum4 : Sum  Inputs=++|
  Sum{5..8} (4 alike) : Sum  Inputs=|+-
  Terminator : Terminator
  Terminator1 : Terminator
  Vcomp LPF : Subsystem
  P_request : Outport
  Q_request : Outport  Port=2
  wires:
  [Vpve] -> Complex to Magnitude/1, Line drop Compensation/2(V)
  Vref/1 -> Saturation8/1
  Gain/1 -> Sum2/1
  [freq] -> Sum5/2
  Complex to Real-Imag/2 -> Q LPF/1(u), Gain/1
  FreqRef/1 -> Saturation9/1
  Multiport Switch1/1 -> Vcomp LPF/1(u)
  Sum2/1 -> Multiport Switch1/2
  Vcomp LPF/1(y) -> Sum/1
  QRef/1 -> Saturation6/1
  Line drop Compensation/1(Ve) -> Multiport Switch1/3
  Pref/1 -> Saturation7/1
  Complex to Real-Imag1/1 -> P  LPF/1(u)
  Gain2/1 -> Saturation2/1
  Saturation2/1 -> Sum4/2
  Sum6/1 -> Gain2/1, Gain1/1
  Multiport Switch2/1 -> P Lag LPF/1(u)
  Gain1/1 -> Saturation1/1
  Constant2/1 -> Multiport Switch/1
  Sum5/1 -> Sum6/1, Saturation4/1
  Saturation1/1 -> Sum4/1
  Sum1/1 -> Multiport Switch/2
  Sum4/1 -> Sum3/2
  Q LPF/1(y) -> Sum1/1
  Gain4/1 -> Meter/1(v)
  Meter/4(freq) -> Gain5/1
  Meter/1(Vpve) -> Scope2/1, [Vpve]
  Gain3/1 -> Meter/2(i)
  Meter/2(ipve) -> Scope2/2, [ipve]
  Meter/3(S) -> Scope2/3, [S]
  [S] -> Complex to Real-Imag/1
  Complex to Real-Imag/1 -> Terminator/1
  [ipve] -> Line drop Compensation/1(I)
  Complex to Magnitude/1 -> [Vmag], Sum2/2  "Ve"
  [S] -> Complex to Real-Imag1/1
  Complex to Real-Imag1/2 -> Terminator1/1
  Vac/1 -> Gain4/1
  Iac/1 -> Gain3/1
  Saturation4/1 -> Sum6/2
  Constant1/1 -> Multiport Switch1/1
  Constant4/1 -> Multiport Switch2/1
  Multiport Switch/1 -> Sum7/1, Saturation5/1
  Saturation5/1 -> Sum7/2
  Sum7/1 -> Saturation/1
  Saturation/1 -> Reactive Power Controller/1(e)
  Reactive Power Controller/1(u) -> Q Lead Lag/1(u)
  Saturation3/1 -> Active Power Controller/1(e), Scope/2
  Gain5/1 -> Scope2/4, [freq]
  Saturation6/1 -> Sum1/2
  Saturation7/1 -> Sum3/1
  Saturation8/1 -> Sum/2
  Saturation9/1 -> Sum5/1
  [Vmag] -> Less Than/1
  Constant/1 -> Less Than/2
  Less Than/1 -> Reactive Power Controller/3(Hold)
  Constant3/1 -> Less Than1/2
  Less Than1/1 -> Scope/4, Active Power Controller/3(Hold)
  [Vmag] -> Scope/3, Less Than1/1
  P  LPF/1(y) -> Sum8/2
  Constant5/1 -> Multiport Switch3/1
  Multiport Switch3/1 -> Saturation3/1
  Sum8/1 -> Multiport Switch3/3
  Constant6/1 -> Multiport Switch3/2
  Sum3/1 -> Saturation10/1
  Active Power Controller/1(u) -> Scope/1, Multiport Switch2/3
  Saturation10/1 -> Multiport Switch2/2, Sum8/1
  [Vpve] -> LVRT_foldback/1(Vpve_pu)  "V_pu_plant"
  Gain6/1 -> Saturation Dynamic/3
  LVRT_foldback/1(limit_pu) -> Gain6/1, Saturation Dynamic/1  "spinout_limit_Vpcc"
  P Lag LPF/1(y) -> Saturation Dynamic/2
  Saturation Dynamic/1 -> P_request/1
  Q Lead Lag/1(y) -> Q_request/1
  Sum/1 -> Multiport Switch/3
  en/1 -> Selector/1
  Selector/1 -> [en]
  [en] -> Reactive Power Controller/2(en)
  [en] -> Active Power Controller/2(en)

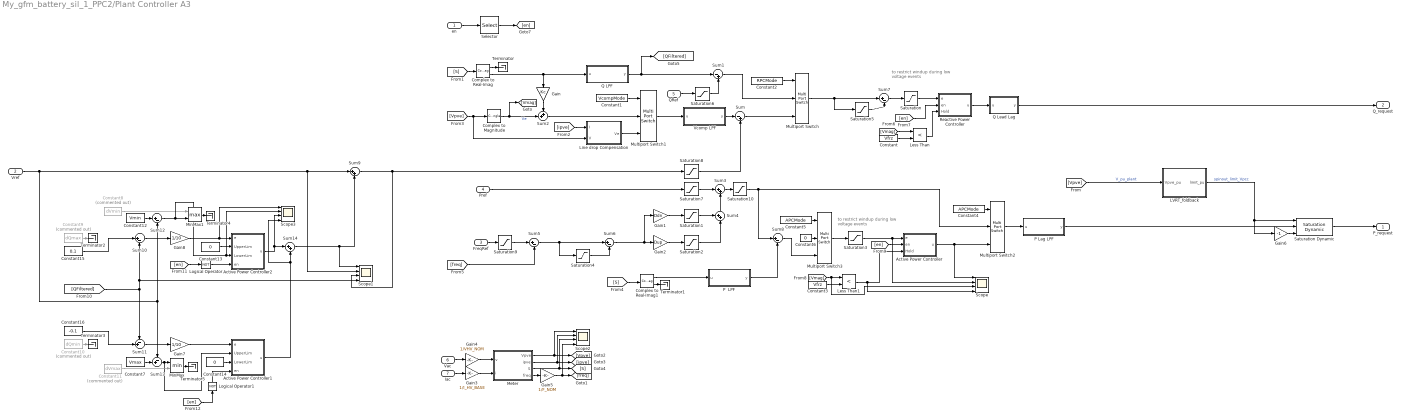
== system My_gfm_battery_sil_1_PPC2/Plant Controller A3 ==
  note: to restrict windup
      | during low voltage events
  note: to restrict windup
      | during low voltage events
  en : Inport
  Vref : Inport  Port=2
  FreqRef : Inport  Port=3
  Pref : Inport  Port=4
  QRef : Inport  Port=5
  Vac : Inport  Port=6
  Iac : Inport  Port=7
  Active Power Controller : Subsystem
  Active Power Controller1 : Subsystem
  Active Power Controller2 : Subsystem
  Complex to Real-Imag : ComplexToRealImag
  Complex to Real-Imag1 : ComplexToRealImag
  Complex to Magnitude : ComplexToMagnitudeAngle  Output=Magnitude
  Constant : Constant  Value=Vfrz
  Constant1 : Constant  Value=VcompMode
  Constant10 : Constant  Commented=on  Value=dQmin
  Constant11 : Constant  Commented=on  Value=dVmax
  Constant12 : Constant  Value=Vmin
  Constant13 : Constant  Value=0
  Constant14 : Constant  Value=0
  Constant15 : Constant  Value=0.1
  Constant16 : Constant  Value=-0.1
  Constant2 : Constant  Value=RPCMode
  Constant3 : Constant  Value=Vfrz
  Constant4 : Constant  Value=APCMode
  Constant5 : Constant  Value=APCMode
  Constant6 : Constant  Value=0
  Constant7 : Constant  Value=Vmax
  Constant8 : Constant  Commented=on  Value=dVmin
  Constant9 : Constant  Commented=on  Value=dQmax
  Gain : Gain  Gain=Kc
  Gain1 : Gain  Gain=Ddn
  Gain2 : Gain  Gain=Dup
  Gain3 : Gain  Gain=1/I_HV_BASE
  Gain4 : Gain  Gain=1/VHV_NOM
  Gain5 : Gain  Gain=1/F_NOM
  Gain6 : Gain  Gain=-1
  Gain7 : Gain  Gain=1/10
  Gain8 : Gain  Gain=1/10
  LVRT_foldback : Subsystem
  Less Than : RelationalOperator  Operator=<  OutDataTypeStr=boolean  RndMeth=Simplest
  Less Than1 : RelationalOperator  Operator=<  OutDataTypeStr=boolean  RndMeth=Simplest
  Line drop Compensation : Subsystem
  Logical Operator : Logic  Operator=NOT  AllPortsSameDT=off  OutDataTypeStr=boolean
  Logical Operator1 : Logic  Operator=NOT  AllPortsSameDT=off  OutDataTypeStr=boolean
  Meter : Subsystem
  MinMax : MinMax  Inputs=2
  MinMax1 : MinMax  Function=max  Inputs=2
  Multiport Switch{,1..3} (4 alike) : MultiPortSwitch  DataPortOrder=Zero-based contiguous  Inputs=2  zeroidx=on
  P  LPF : Subsystem
  P Lag LPF : Subsystem
  Q LPF : Subsystem
  Q Lead Lag : Subsystem
  Reactive Power Controller : Subsystem
  Saturation : Saturate  UpperLimit=emax  LowerLimit=emin
  Saturation Dynamic : simulink/Discontinuities/Saturation Dynamic  OutMin=[]  OutMax=[]  OutDataTypeStr=Inherit: Same as second input  OutDataType=fixdt(1, 16)  OutScaling=2^-10  DoSatur=off
  Saturation1 : Saturate  UpperLimit=0  LowerLimit=-inf
  Saturation10 : Saturate  UpperLimit=PRefmax  LowerLimit=PRefmin
  Saturation2 : Saturate  UpperLimit=inf  LowerLimit=0
  Saturation3 : Saturate  UpperLimit=femax  LowerLimit=femin
  Saturation4 : Saturate  UpperLimit=fdbd1  LowerLimit=fdbd2
  Saturation5 : Saturate  UpperLimit=db1  LowerLimit=-db1
  Saturation6 : Saturate  UpperLimit=QRefmax  LowerLimit=QRefmin
  Saturation7 : Saturate  UpperLimit=PRefmax  LowerLimit=PRefmin
  Saturation8 : Saturate  UpperLimit=Vmax  LowerLimit=Vmin
  Saturation9 : Saturate  UpperLimit=Fmax  LowerLimit=Fmin
  Scope{,1..3} (4 alike) : Scope  NumInputPorts=4
  Selector : Selector  InputPortWidth=3  IndexOptions=Index vector (dialog)  Indices=[1]  OutputSizes=1
  Sum : Sum  Inputs=|-+
  Sum1 : Sum  Inputs=|-+
  Sum{5..8,10,12} (6 alike) : Sum  Inputs=|+-
  Sum11 : Sum  Inputs=-+|
  Sum13 : Sum  Inputs=-+|
  Sum14 : Sum  Inputs=|++
  Sum2 : Sum  Inputs=++|
  Sum3 : Sum  Inputs=|++
  Sum4 : Sum  Inputs=++|
  Sum9 : Sum  Inputs=|++
  Terminator{,1..5} (6 alike) : Terminator
  Vcomp LPF : Subsystem
  P_request : Outport
  Q_request : Outport  Port=2
  wires:
  [Vpve] -> Complex to Magnitude/1, Line drop Compensation/2(V)
  Sum9/1 -> Saturation8/1, Scope1/3
  Gain/1 -> Sum2/1
  [freq] -> Sum5/2
  Complex to Real-Imag/2 -> Q LPF/1(u), Gain/1
  FreqRef/1 -> Saturation9/1
  Multiport Switch1/1 -> Vcomp LPF/1(u)
  Sum2/1 -> Multiport Switch1/2
  Vcomp LPF/1(y) -> Sum/1
  QRef/1 -> Saturation6/1
  Line drop Compensation/1(Ve) -> Multiport Switch1/3
  Pref/1 -> Saturation7/1
  Complex to Real-Imag1/1 -> P  LPF/1(u)
  Gain2/1 -> Saturation2/1
  Saturation2/1 -> Sum4/2
  Sum6/1 -> Gain2/1, Gain1/1
  Multiport Switch2/1 -> P Lag LPF/1(u)
  Gain1/1 -> Saturation1/1
  Constant2/1 -> Multiport Switch/1
  Sum5/1 -> Sum6/1, Saturation4/1
  Saturation1/1 -> Sum4/1
  Sum1/1 -> Multiport Switch/2
  Sum4/1 -> Sum3/2
  Q LPF/1(y) -> [QFiltered], Sum1/1
  Gain4/1 -> Meter/1(v)
  Meter/4(freq) -> Gain5/1
  Meter/1(Vpve) -> Scope2/1, [Vpve]
  Gain3/1 -> Meter/2(i)
  Meter/2(ipve) -> Scope2/2, [ipve]
  Meter/3(S) -> Scope2/3, [S]
  [S] -> Complex to Real-Imag/1
  Complex to Real-Imag/1 -> Terminator/1
  [ipve] -> Line drop Compensation/1(I)
  Complex to Magnitude/1 -> [Vmag], Sum2/2  "Ve"
  [S] -> Complex to Real-Imag1/1
  Complex to Real-Imag1/2 -> Terminator1/1
  Vac/1 -> Gain4/1
  Iac/1 -> Gain3/1
  Saturation4/1 -> Sum6/2
  Constant1/1 -> Multiport Switch1/1
  Constant4/1 -> Multiport Switch2/1
  Multiport Switch/1 -> Sum7/1, Saturation5/1
  Saturation5/1 -> Sum7/2
  Sum7/1 -> Saturation/1
  Saturation/1 -> Reactive Power Controller/1(e)
  Reactive Power Controller/1(u) -> Q Lead Lag/1(u)
  Saturation3/1 -> Active Power Controller/1(e), Scope/2
  Gain5/1 -> Scope2/4, [freq]
  Saturation6/1 -> Sum1/2
  Saturation7/1 -> Sum3/1
  Saturation8/1 -> Sum/2
  Saturation9/1 -> Sum5/1
  [Vmag] -> Less Than/1
  Constant/1 -> Less Than/2
  Less Than/1 -> Reactive Power Controller/3(Hold)
  Constant3/1 -> Less Than1/2
  Less Than1/1 -> Scope/4, Active Power Controller/3(Hold)
  [Vmag] -> Scope/3, Less Than1/1
  P  LPF/1(y) -> Sum8/2
  Constant5/1 -> Multiport Switch3/1
  Multiport Switch3/1 -> Saturation3/1
  Sum8/1 -> Multiport Switch3/3
  Constant6/1 -> Multiport Switch3/2
  Sum3/1 -> Saturation10/1
  Active Power Controller/1(u) -> Scope/1, Multiport Switch2/3
  Saturation10/1 -> Multiport Switch2/2, Sum8/1
  [Vpve] -> LVRT_foldback/1(Vpve_pu)  "V_pu_plant"
  Gain6/1 -> Saturation Dynamic/3
  LVRT_foldback/1(limit_pu) -> Gain6/1, Saturation Dynamic/1  "spinout_limit_Vpcc"
  P Lag LPF/1(y) -> Saturation Dynamic/2
  Saturation Dynamic/1 -> P_request/1
  Q Lead Lag/1(y) -> Q_request/1
  Sum/1 -> Multiport Switch/3
  en/1 -> Selector/1
  Selector/1 -> [en]
  [en] -> Reactive Power Controller/2(en)
  [en] -> Active Power Controller/2(en)
  MinMax/1 -> Terminator5/1
  MinMax1/1 -> Terminator4/1
  Constant7/1 -> Sum13/2
  Constant9/1 -> Terminator2/1
  Sum13/1 -> Active Power Controller1/2(UpperLim), MinMax/1
  Constant8/1 -> MinMax1/1
  Sum14/1 -> Scope1/1, Sum9/2
  Constant14/1 -> Active Power Controller1/3(LowerLim)
  Constant15/1 -> Sum10/1
  Constant11/1 -> MinMax/2
  Gain8/1 -> Active Power Controller2/1(e), Scope3/1
  Active Power Controller1/1(u) -> Scope3/4, Sum14/2
  [QFiltered] -> Scope1/4, Sum10/2, Sum11/1
  Active Power Controller2/1(u) -> Scope3/3, Sum14/1
  Constant13/1 -> Active Power Controller2/2(UpperLim)
  Constant12/1 -> Sum12/1
  Sum11/1 -> Gain7/1
  Sum10/1 -> Gain8/1
  Gain7/1 -> Active Power Controller1/1(e)
  Constant16/1 -> Sum11/2
  Vref/1 -> Scope1/2, Sum9/1, Sum13/1, Sum12/2
  Constant10/1 -> Terminator3/1
  [en] -> Logical Operator/1
  [en] -> Logical Operator1/1
  Sum12/1 -> Scope3/2, Active Power Controller2/3(LowerLim), MinMax1/2
  Logical Operator/1 -> Active Power Controller2/4(en)
  Logical Operator1/1 -> Active Power Controller1/4(en)
